simulink model "membrane_convergence"  (R2025b)
settings: Solver=VariableStepAuto  StartTime=0.0  StopTime=1000000  RelTol=1e-3
undefined symbols (not defined in the file or in its folder): N_units
libraries: customization_lib x5, nesl_utility x1
settings Model: Creator=degoede  LastModifiedBy=degoede
settings SimscapeCC: SimscapeLogType=all

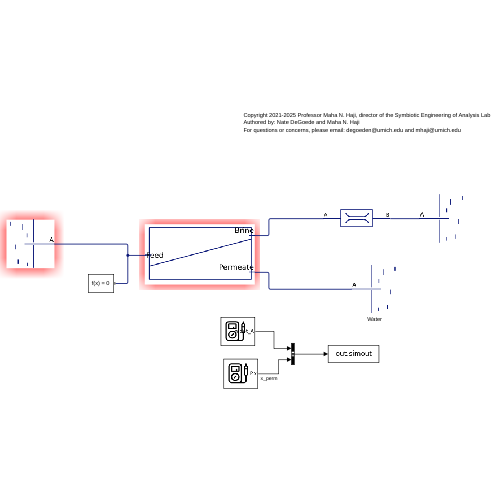
[thumbnail: Simulink's stored preview of the top-level diagram]
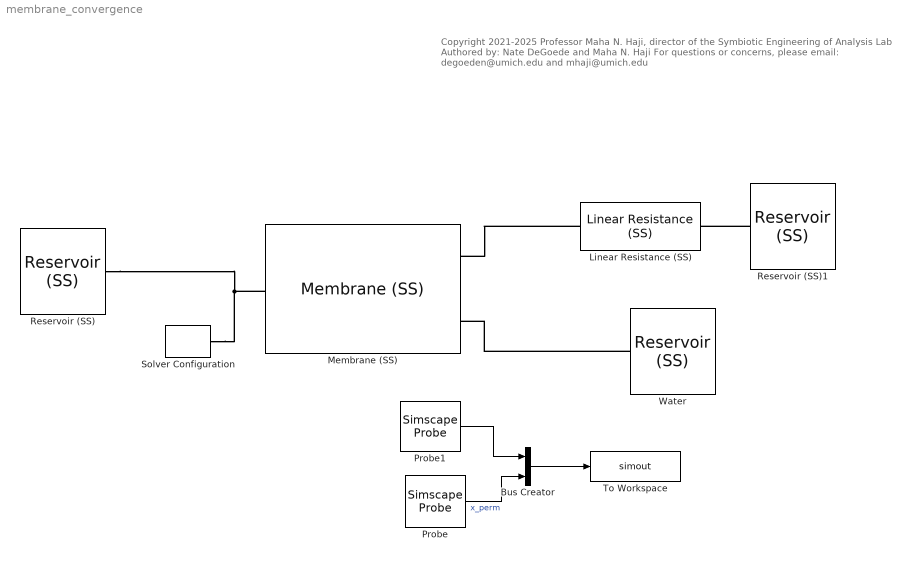
== system membrane_convergence ==
  note: Copyright 2021-2025 Professor Maha N. Haji, director of the Symbiotic Engineering of Analysis Lab
      | Authored by: Nate DeGoede and Maha N. Haji
      | For questions or concerns, please email: degoeden@umich.edu and mhaji@umich.edu
  Bus Creator : BusCreator  Inputs=2
  Linear Resistance (SS) : customization_lib/solution/elements/Linear Resistance (SS)  R=6423000000 Pa*s/m^3  area=0.01 m^2
      settings: SourceProductName=Customization  InternalSimscapePortConfiguration="{\"Bottom\":[],\"Left\":[{\"id\":\"A\",\"label\":\"A\",\"type\":\"customization.solution.solution\"}],\"Right\":[{\"id\":\"B\",\"label\":\"B\",\"type\":\"customization.solution.solution\"}],\"Top\":[]}"
  Membrane (SS) : customization_lib/membranes/Membrane (SS)  A_w=A_w m^3/(N*s)  B_s=B_s m/s  A_m=A_m m^2  length=length m  D_feed=D_feed mm  area_feed=area_feed mm^2  D_perm=D_perm mm  N=N_units  P0_feed=P_feed MPa  P0_perm=0.101 MPa  x0_feed=x_feed kg/m^3  x0_perm=0 kg/m^3
      settings: SourceProductName=Customization  InternalSimscapePortConfiguration="{\"Bottom\":[],\"Left\":[{\"id\":\"F\",\"label\":\"Feed\",\"type\":\"customization.solution.solution\"}],\"Right\":[{\"id\":\"B\",\"label\":\"Brine\",\"type\":\"customization.solution.solution\"},{\"id\":\"P\",\"label\":\"Permeate\",\"type\":\"customization.solution.solution\"}],\"Top\":[]}"
  Probe : SimscapeProbe  BoundBlock=22  Variables="{\"P.x\":{\"Probing\":\"ON\"}}"
  Probe1 : SimscapeProbe  BoundBlock=18  Variables="{\"mdot_A\":{\"Probing\":\"ON\"}}"
  Reservoir (SS) : customization_lib/solution/elements/Reservoir (SS)  pressure_spec=foundation.enum.pressure_spec.specified  reservoir_pressure=P_feed MPa  reservoir_temperature=293.15 K  reservoir_concentration=x_feed kg/m^3  area=1 cm^2
      settings: SourceProductName=Customization  InternalSimscapePortConfiguration="{\"Bottom\":[],\"Left\":[{\"id\":\"A\",\"label\":\"A\",\"type\":\"customization.solution.solution\"}],\"Right\":[],\"Top\":[]}"
  Reservoir (SS)1 : customization_lib/solution/elements/Reservoir (SS)  pressure_spec=foundation.enum.pressure_spec.atmospheric  reservoir_pressure=0.101325 MPa  reservoir_temperature=293.15 K  reservoir_concentration=50 kg/m^3  area=27 mm^2
      settings: SourceProductName=Customization  InternalSimscapePortConfiguration="{\"Bottom\":[],\"Left\":[{\"id\":\"A\",\"label\":\"A\",\"type\":\"customization.solution.solution\"}],\"Right\":[],\"Top\":[]}"
  Solver Configuration : nesl_utility/Solver Configuration  PhysicalDomain=network_engine_domain  SubClassName=solver  LeftPortType=input  RightPortType=generic  Tones=[]  Harmonics=[]  SimulateNoise=off  Profile=off  UseLocalSampling=off  EnableSwitchedLinearOptims=on  FrequencyDomain=off  UseCCode=off  RelTol=0.001  AbsTol=0.001  MinStep=1e-09  ToWorkspace=off  RevertToSquareIcSolve=off  NumHomotopyIterations=100  PhasorMode=off  PhasorModeNumHarmonics=1  ConsistencySolver=NEWTON_XTOL_AFTER_FTOL  IndexReductionMethod=DerivativeReplacement  DoDC=off  ResidualTolerance=1e-09  ConsistencyTolSource=GLOBAL  ConsistencyAbsTol=0.001  ConsistencyRelTol=0.001  ConsistencyTolFactor=0.001  UseLocalSolver=off  LocalSolverChoice=NE_BACKWARD_EULER_ADVANCER  ResolveIndetEquations=on  FunctionEvalNumThread=1  LocalSolverSampleTime=0.001  DoFixedCost=off  MaxNonlinIter=3  MaxModeIter=2  ComputeImpulses=off  ImpulseIterations=2  LinearAlgebra=auto  LinearAlgebraNumThread=0  EquationFormulation=NE_TIME_EF  DelaysMemoryBudget=1024  AutomaticFiltering=off  FilteringTimeConstant=0.001  PartitionStorageMethod=AS_NEEDED  PartitionMemoryBudget=1024  PartitionMethod=ROBUST  MultibodyUseLocalSolver=off  MultibodyLocalSolverChoice=ODE1  MultibodyLocalSolverSampleTime=0.001
  To Workspace : ToWorkspace  VariableName=simout  SaveFormat=Timeseries  SampleTime=-1
  Water : customization_lib/solution/elements/Reservoir (SS)  pressure_spec=foundation.enum.pressure_spec.atmospheric  reservoir_pressure=0.101325 MPa  reservoir_temperature=293.15 K  reservoir_concentration=0 kg/m^3  area=1 cm^2
      settings: SourceProductName=Customization  InternalSimscapePortConfiguration="{\"Bottom\":[],\"Left\":[{\"id\":\"A\",\"label\":\"A\",\"type\":\"customization.solution.solution\"}],\"Right\":[],\"Top\":[]}"
  wires:
  Probe/1 -> Bus Creator/2  "x_perm"
  Bus Creator/1 -> To Workspace/1
  Probe1/1 -> Bus Creator/1
  connections:
  Solver Configuration/RConn1 -- Membrane (SS)/LConn1 -- Reservoir (SS)/LConn1
  Linear Resistance (SS)/LConn1 -- Membrane (SS)/RConn1
  Water/LConn1 -- Membrane (SS)/RConn2
  Reservoir (SS)1/LConn1 -- Linear Resistance (SS)/RConn1
